simulink model "ACC4_FFNN_trainbfg_15_15_15_ep_100_Nor_20250527"  (R2021a)
settings: Solver=FixedStepAuto  StartTime=0.0  StopTime=T  RelTol=1e-3
undefined symbols (not defined in the file or in its folder): t_gap, Ts, v0_ego, v0_lead, v_set, x0_ego, x0_lead, x_gain, x_offset, y_gain, y_offset
libraries: neural x50
(part 2 of 2)

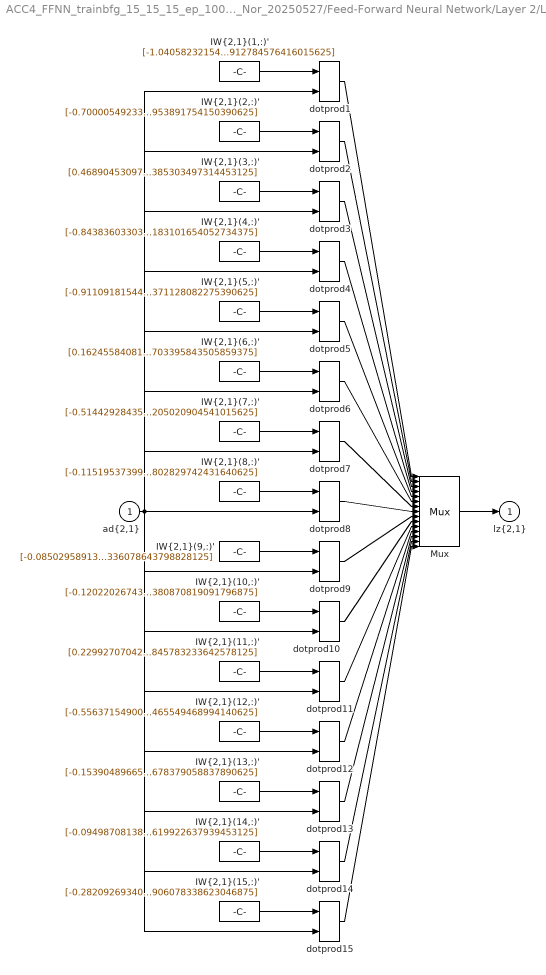
== system ACC4_FFNN_trainbfg_15_15_15_ep_100_Nor_20250527/Feed-Forward Neural Network/Layer 2/LW{2,1} ==
  "ad{2,1}" : Inport  PortDimensions=15
      mask Display: e = 0.06;c1 = [120 230 180]/255;c2 = ([120 230 180]+0)/(256+128);c3 = ([120 230 180]+128)/(256+128);patch([0 1 1 0],[0 0 1 1],c1);patch([0 1 1 1-e 1-e 0+e],[0 0 1 1-e 0+e 0+e],c2);patch([0 0 1 1-e 0+e 0+e],[0 1 1 1-e 1-e 0+e],c3);plot([0 1 1 0 0],[0 0 1 1 0]);
  "IW{2,1}(1,:)'" : Constant  Value=[-1.0405823215489833355462678809999488294124603271484375;-0.9608271683105680249781244128826074302196502685546875;0.5476392940007086540532554863602854311466217041015625;-0.1860903257221864226522711760480888187885284423828125;0.70133754923509872281073285193997435271739959716796875;-0.54431412858791627940036050858907401561737060546875;0.5380581706717924017624454791075550019741058349609375;-0.9009348419158775822523921306128613650798797607421875;-0.7521354448038597428904949993011541664600372314453125;0.241917287870616615208518851432017982006072998046875;-0.7321374980240575869316899115801788866519927978515625;-0.6457849324217816988635831876308657228946685791015625;-0.64376602939558436045075495712808333337306976318359375;-0.63161180496894697711240951321087777614593505859375;0.516510433268904112225072822184301912784576416015625]
      mask Display: e = 0.06;c1 = [120 150 230]/255;c2 = ([120 150 230]+0)/383;c3 = ([120 150 230]+128)/383;patch([0 1 1 0],[0 0 1 1],c1);patch([0 1 1 1-e 1-e 0+e],[0 0 1 1-e 0+e 0+e],c2);patch([0 0 1 1-e 0+e 0+e],[0 1 1 1-e 1-e 0+e],c3);plot([0 1 1 0 0],[0 0 1 1 0]);disp('weights');
  "IW{2,1}(10,:)'" : Constant  Value=[-0.120220267431918659273293314981856383383274078369140625;0.5302574432542292992565080567146651446819305419921875;1.0844112018206886194349181096185930073261260986328125;0.3573046096003764660054002888500690460205078125;0.73117639412220347683302179575548507273197174072265625;-0.75418929339658602462037606528610922396183013916015625;-0.581189831958130564970588238793425261974334716796875;-0.4362662882391401542037101535242982208728790283203125;-0.588048968935513283184945976245217025279998779296875;0.968796624481943258189176049199886620044708251953125;0.6844132248386689543195871010539121925830841064453125;-0.3617435753298094969210296767414547502994537353515625;-0.00872169059706992023939253755315803573466837406158447265625;-0.1165558858711521761364338090061210095882415771484375;0.36089370267177389717261348778265528380870819091796875]
      mask Display: e = 0.06;c1 = [120 150 230]/255;c2 = ([120 150 230]+0)/383;c3 = ([120 150 230]+128)/383;patch([0 1 1 0],[0 0 1 1],c1);patch([0 1 1 1-e 1-e 0+e],[0 0 1 1-e 0+e 0+e],c2);patch([0 0 1 1-e 0+e 0+e],[0 1 1 1-e 1-e 0+e],c3);plot([0 1 1 0 0],[0 0 1 1 0]);disp('weights');
  "IW{2,1}(11,:)'" : Constant  Value=[0.2299270704222209360523265786468982696533203125;-0.1990641851978147414126141256929258815944194793701171875;0.0157493935539519784583273320777152548544108867645263671875;-0.0096459618206787833827320355339907109737396240234375;0.225314821626530104037300361596862785518169403076171875;0.1739138266543526489815718605314032174646854400634765625;0.1045826830775500315695580866304226219654083251953125;0.07719335609068078696282100281678140163421630859375;0.8958662425863372913426019295002333819866180419921875;0.7178776333677323595594543803599663078784942626953125;0.118065089977390069719831444672308862209320068359375;-0.23311728925552344104943358615855686366558074951171875;0.7705319447275733590885238299961201846599578857421875;-0.97343359906549498106187456869520246982574462890625;0.043267329398776928350844883652825956232845783233642578125]
      mask Display: e = 0.06;c1 = [120 150 230]/255;c2 = ([120 150 230]+0)/383;c3 = ([120 150 230]+128)/383;patch([0 1 1 0],[0 0 1 1],c1);patch([0 1 1 1-e 1-e 0+e],[0 0 1 1-e 0+e 0+e],c2);patch([0 0 1 1-e 0+e 0+e],[0 1 1 1-e 1-e 0+e],c3);plot([0 1 1 0 0],[0 0 1 1 0]);disp('weights');
  "IW{2,1}(12,:)'" : Constant  Value=[-0.556371549001076548535138499573804438114166259765625;0.6163768674988137075132499376195482909679412841796875;0.454735929886855572146231452279607765376567840576171875;-0.6205791879648396847102276296936906874179840087890625;0.9799003554114114056261541918502189218997955322265625;0.10021329629212542833283094978469307534396648406982421875;0.25976677012884241690926501178182661533355712890625;0.390326078888663996480090645491145551204681396484375;-0.835857585804548275376646415679715573787689208984375;0.571117978530061076725132807041518390178680419921875;0.70819989854688625285916714346967637538909912109375;-0.246601959183730790048372227829531766474246978759765625;-0.94243259499025811010142206214368343353271484375;0.794382701947144109766441033571027219295501708984375;-0.89798245506530138815293184961774386465549468994140625]
      mask Display: e = 0.06;c1 = [120 150 230]/255;c2 = ([120 150 230]+0)/383;c3 = ([120 150 230]+128)/383;patch([0 1 1 0],[0 0 1 1],c1);patch([0 1 1 1-e 1-e 0+e],[0 0 1 1-e 0+e 0+e],c2);patch([0 0 1 1-e 0+e 0+e],[0 1 1 1-e 1-e 0+e],c3);plot([0 1 1 0 0],[0 0 1 1 0]);disp('weights');
  "IW{2,1}(13,:)'" : Constant  Value=[-0.153904896659829371063921144013875164091587066650390625;0.5090717228071948152745562765630893409252166748046875;-0.29697183815985350729960146054509095847606658935546875;-0.0099883500195583341252358877682127058506011962890625;0.05536005484219876093821000040406943298876285552978515625;0.1251542077321984580695612976342090405523777008056640625;-0.9360179684748661799176261411048471927642822265625;-0.0017679730348210132007125139352865517139434814453125;-0.7885811468365571119676360467565245926380157470703125;0.0267548371751498148540804322692565619945526123046875;-0.3042416113454777804037121313740499317646026611328125;0.261979220371351961826889009898877702653408050537109375;0.2643737023407515263073719324893318116664886474609375;-0.606683617264736074758957329322583973407745361328125;-0.95567583042114601088456993238651193678379058837890625]
      mask Display: e = 0.06;c1 = [120 150 230]/255;c2 = ([120 150 230]+0)/383;c3 = ([120 150 230]+128)/383;patch([0 1 1 0],[0 0 1 1],c1);patch([0 1 1 1-e 1-e 0+e],[0 0 1 1-e 0+e 0+e],c2);patch([0 0 1 1-e 0+e 0+e],[0 1 1 1-e 1-e 0+e],c3);plot([0 1 1 0 0],[0 0 1 1 0]);disp('weights');
  "IW{2,1}(14,:)'" : Constant  Value=[-0.0949870813828463667061186015416751615703105926513671875;-0.230612941886796762869238364146440289914608001708984375;-1.0507342618771271514077625397476367652416229248046875;-0.7047835560466226834108738330542109906673431396484375;-0.04152563470139190859864442018078989349305629730224609375;0.58730051068405131342586855680565349757671356201171875;0.2294268382342810053131643144297413527965545654296875;0.071602111502226506445367704145610332489013671875;-0.7159177561920035959275310233351774513721466064453125;-0.644795078988269931841159632313065230846405029296875;-0.1079467038897943265141066149226389825344085693359375;0.48203925309316908442980320614879019558429718017578125;0.33818146513637958872067201809841208159923553466796875;-0.8132589664898139947268873584107495844364166259765625;0.478036667924507885363283321566996164619922637939453125]
      mask Display: e = 0.06;c1 = [120 150 230]/255;c2 = ([120 150 230]+0)/383;c3 = ([120 150 230]+128)/383;patch([0 1 1 0],[0 0 1 1],c1);patch([0 1 1 1-e 1-e 0+e],[0 0 1 1-e 0+e 0+e],c2);patch([0 0 1 1-e 0+e 0+e],[0 1 1 1-e 1-e 0+e],c3);plot([0 1 1 0 0],[0 0 1 1 0]);disp('weights');
  "IW{2,1}(15,:)'" : Constant  Value=[-0.2820926934058338719779612802085466682910919189453125;-0.55856947057804762213351068567135371267795562744140625;-0.551556482284416116357306236750446259975433349609375;-0.890051706187623636878925026394426822662353515625;0.60240233369460483014989904404501430690288543701171875;0.96460639263537995002906200170400552451610565185546875;-0.2751770754538946928136056158109568059444427490234375;-0.10963366940791541281896570581011474132537841796875;-0.667079118247158486809667010675184428691864013671875;-0.2028210065283138074931912342435680329799652099609375;-0.891521031117740836435814344440586864948272705078125;-0.799556919609016869543438588152639567852020263671875;0.12267233388357355605702281309277168475091457366943359375;-0.3852662008241598545765782546368427574634552001953125;0.6905806241987288984773840638808906078338623046875]
      mask Display: e = 0.06;c1 = [120 150 230]/255;c2 = ([120 150 230]+0)/383;c3 = ([120 150 230]+128)/383;patch([0 1 1 0],[0 0 1 1],c1);patch([0 1 1 1-e 1-e 0+e],[0 0 1 1-e 0+e 0+e],c2);patch([0 0 1 1-e 0+e 0+e],[0 1 1 1-e 1-e 0+e],c3);plot([0 1 1 0 0],[0 0 1 1 0]);disp('weights');
  "IW{2,1}(2,:)'" : Constant  Value=[-0.7000054923366338943679920703289099037647247314453125;-0.3382842395718579364682909726980142295360565185546875;0.8986078236995937995601479997276328504085540771484375;0.4974114364313828584585053249611519277095794677734375;0.1211190547097695802136740894638933241367340087890625;-0.003811417607220590753058786503970623016357421875;0.162892975750795532263737186440266668796539306640625;-0.0208600216453564968333012075163424015045166015625;-0.0192854130639636967003980316803790628910064697265625;0.147419529682396355241280616610310971736907958984375;-0.9382209025100969324029165363754145801067352294921875;0.325616123921948830144401654251851141452789306640625;-0.2807301730358393587749787911889143288135528564453125;0.19442270067570976976867314078845083713531494140625;-0.7966612127504897333807321047061122953891754150390625]
      mask Display: e = 0.06;c1 = [120 150 230]/255;c2 = ([120 150 230]+0)/383;c3 = ([120 150 230]+128)/383;patch([0 1 1 0],[0 0 1 1],c1);patch([0 1 1 1-e 1-e 0+e],[0 0 1 1-e 0+e 0+e],c2);patch([0 0 1 1-e 0+e 0+e],[0 1 1 1-e 1-e 0+e],c3);plot([0 1 1 0 0],[0 0 1 1 0]);disp('weights');
  "IW{2,1}(3,:)'" : Constant  Value=[0.46890453097095063927923774826922453939914703369140625;-0.1600608568250439234237347818634589202702045440673828125;-0.12399845995805358622732228468521498143672943115234375;0.6511676315723111674316214703139849007129669189453125;0.85938165041460357063130004462436772882938385009765625;0.967936511731725790497193884220905601978302001953125;0.856626124628375951175485170097090303897857666015625;-0.6149792078758504754176783535513095557689666748046875;0.7059963106816324884817959173233248293399810791015625;-0.8958442194282607573541099554859101772308349609375;0.8782834121390958870279064285568892955780029296875;-0.206000980504430941664395504631102085113525390625;-0.77406206789949927316030198198859579861164093017578125;-0.4001260198204221740780894833733327686786651611328125;0.82207842077581905204652912289020605385303497314453125]
      mask Display: e = 0.06;c1 = [120 150 230]/255;c2 = ([120 150 230]+0)/383;c3 = ([120 150 230]+128)/383;patch([0 1 1 0],[0 0 1 1],c1);patch([0 1 1 1-e 1-e 0+e],[0 0 1 1-e 0+e 0+e],c2);patch([0 0 1 1-e 0+e 0+e],[0 1 1 1-e 1-e 0+e],c3);plot([0 1 1 0 0],[0 0 1 1 0]);disp('weights');
  "IW{2,1}(4,:)'" : Constant  Value=[-0.84383603303488075031424386907019652426242828369140625;-0.45965468593376723749344137104344554245471954345703125;0.0104593103155407908533280902929618605412542819976806640625;0.579926059889061651375641304184682667255401611328125;0.3933344011104551452007171974400989711284637451171875;-0.08418835848849438863172878200202831067144870758056640625;0.1601807315168832790419628508971072733402252197265625;-0.753832504908109601871046834276057779788970947265625;0.7478548117234666836594669803162105381488800048828125;0.862402769216499276438980814418755471706390380859375;-0.3973878708272156057290658281999640166759490966796875;0.6115292870810014047577851670212112367153167724609375;-0.11578681594154351108816314308569417335093021392822265625;-0.7317541343426352540291190962307155132293701171875;-0.417232981103956512836106185204698704183101654052734375]
      mask Display: e = 0.06;c1 = [120 150 230]/255;c2 = ([120 150 230]+0)/383;c3 = ([120 150 230]+128)/383;patch([0 1 1 0],[0 0 1 1],c1);patch([0 1 1 1-e 1-e 0+e],[0 0 1 1-e 0+e 0+e],c2);patch([0 0 1 1-e 0+e 0+e],[0 1 1 1-e 1-e 0+e],c3);plot([0 1 1 0 0],[0 0 1 1 0]);disp('weights');
  "IW{2,1}(5,:)'" : Constant  Value=[-0.9110918154435230231769082820392213761806488037109375;-0.6058924038090884867102658972726203501224517822265625;-0.122710034826088776327424056944437325000762939453125;-0.3629515092020156874497160970349796116352081298828125;0.165581930351680117752266596653498709201812744140625;0.6903563701080732695203323601162992417812347412109375;-0.96603412332547744512112330994568765163421630859375;-0.5890116581846402965538800344802439212799072265625;-0.45941133541460477118789640371687710285186767578125;0.457323363356542333946208600536920130252838134765625;-0.408932331049287167701322687207721173763275146484375;-0.763689603106578740465693044825457036495208740234375;-0.3283020506461509224749306667945347726345062255859375;-0.574796933282314181923311480204574763774871826171875;-0.4053063682241566656472286922507919371128082275390625]
      mask Display: e = 0.06;c1 = [120 150 230]/255;c2 = ([120 150 230]+0)/383;c3 = ([120 150 230]+128)/383;patch([0 1 1 0],[0 0 1 1],c1);patch([0 1 1 1-e 1-e 0+e],[0 0 1 1-e 0+e 0+e],c2);patch([0 0 1 1-e 0+e 0+e],[0 1 1 1-e 1-e 0+e],c3);plot([0 1 1 0 0],[0 0 1 1 0]);disp('weights');
  "IW{2,1}(6,:)'" : Constant  Value=[0.162455840818920560497673477584612555801868438720703125;0.642616637081111274909517305786721408367156982421875;0.350996130621946067495997567675658501684665679931640625;0.0681282547414527872575717992731370031833648681640625;0.63079436754187601099630455792066641151905059814453125;0.253691470335771274147163012457895092666149139404296875;-0.7582808578028836787865429869270883500576019287109375;-0.7069701787702202810947937905439175665378570556640625;-0.5830772824973724510755346273072063922882080078125;0.4756833075951802936032208890537731349468231201171875;-0.3341274363276494074881384221953339874744415283203125;0.7989442886824651424149124068208038806915283203125;-0.800060224384415707987727728323079645633697509765625;0.789883350881628754081020815647207200527191162109375;-0.95452869287727748481842127148411236703395843505859375]
      mask Display: e = 0.06;c1 = [120 150 230]/255;c2 = ([120 150 230]+0)/383;c3 = ([120 150 230]+128)/383;patch([0 1 1 0],[0 0 1 1],c1);patch([0 1 1 1-e 1-e 0+e],[0 0 1 1-e 0+e 0+e],c2);patch([0 0 1 1-e 0+e 0+e],[0 1 1 1-e 1-e 0+e],c3);plot([0 1 1 0 0],[0 0 1 1 0]);disp('weights');
  "IW{2,1}(7,:)'" : Constant  Value=[-0.5144292843580762220057067679590545594692230224609375;-0.140157181233467209580112466937862336635589599609375;0.537708504859229829975220127380453050136566162109375;-0.82009864245883790090374532155692577362060546875;0.7580278091943555285325828663189895451068878173828125;0.17197407165295164332974309218116104602813720703125;0.725421437399339286145050209597684442996978759765625;-0.621855651054772362584799338947050273418426513671875;0.1299591414764023067363041263888590037822723388671875;-0.8731909986143635560296161202131770551204681396484375;-0.065863625942295112025703929248265922069549560546875;0.0799641980758583059696320560760796070098876953125;-0.582106652013729242156614418490789830684661865234375;-0.8570943744259109653427231023670174181461334228515625;-0.40351205622447228194005219847895205020904541015625]
      mask Display: e = 0.06;c1 = [120 150 230]/255;c2 = ([120 150 230]+0)/383;c3 = ([120 150 230]+128)/383;patch([0 1 1 0],[0 0 1 1],c1);patch([0 1 1 1-e 1-e 0+e],[0 0 1 1-e 0+e 0+e],c2);patch([0 0 1 1-e 0+e 0+e],[0 1 1 1-e 1-e 0+e],c3);plot([0 1 1 0 0],[0 0 1 1 0]);disp('weights');
  "IW{2,1}(8,:)'" : Constant  Value=[-0.1151953739961133482694322083261795341968536376953125;0.7755419085127075451424616403528489172458648681640625;-0.665492909010556576987482912954874336719512939453125;-0.776588511613593102111963162315078079700469970703125;0.9778232321591782127967462656670249998569488525390625;-0.5065309480280502096860573146841488778591156005859375;-0.031406977575795025359184364788234233856201171875;-0.9146951781777132861606105507235042750835418701171875;0.2806236503255161718328736242256127297878265380859375;0.720881126076463818463935240288265049457550048828125;0.2963968129323142353115372316096909344196319580078125;0.413834838645525504574607111862860620021820068359375;0.8103071180089280733938039702479727566242218017578125;-0.5150268821265611141058116118074394762516021728515625;-0.90729747020363848974966458627022802829742431640625]
      mask Display: e = 0.06;c1 = [120 150 230]/255;c2 = ([120 150 230]+0)/383;c3 = ([120 150 230]+128)/383;patch([0 1 1 0],[0 0 1 1],c1);patch([0 1 1 1-e 1-e 0+e],[0 0 1 1-e 0+e 0+e],c2);patch([0 0 1 1-e 0+e 0+e],[0 1 1 1-e 1-e 0+e],c3);plot([0 1 1 0 0],[0 0 1 1 0]);disp('weights');
  "IW{2,1}(9,:)'" : Constant  Value=[-0.08502958913522730421963302660515182651579380035400390625;-0.2182372384019506117436293379796552471816539764404296875;0.309604443959900610394697650917805731296539306640625;-0.727414902123402651312744637834839522838592529296875;-0.99895538327737021244701054456527344882488250732421875;0.045954384797662332917678185140175628475844860076904296875;0.6897113491525264095116654061712324619293212890625;0.270395833719764056013445951975882053375244140625;-0.16594209671422799345918974722735583782196044921875;0.8688102379224267313162499704048968851566314697265625;-0.9495436370139274107060600726981647312641143798828125;0.77107377246475639065437235331046395003795623779296875;0.15514524096584392243158845303696580231189727783203125;-0.892491215582572383624437861726619303226470947265625;-0.1202330084681953181746649761407752521336078643798828125]
      mask Display: e = 0.06;c1 = [120 150 230]/255;c2 = ([120 150 230]+0)/383;c3 = ([120 150 230]+128)/383;patch([0 1 1 0],[0 0 1 1],c1);patch([0 1 1 1-e 1-e 0+e],[0 0 1 1-e 0+e 0+e],c2);patch([0 0 1 1-e 0+e 0+e],[0 1 1 1-e 1-e 0+e],c3);plot([0 1 1 0 0],[0 0 1 1 0]);disp('weights');
  Mux : Mux  Inputs=15
      mask Display: e = 0.06;c1 = [120 150 230]/255;c2 = ([120 150 230]+0)/383;c3 = ([120 150 230]+128)/383;patch([0 1 1 0],[0 0 1 1],c1);patch([0 1 1 1-e 1-e 0+e],[0 0 1 1-e 0+e 0+e],c2);patch([0 0 1 1-e 0+e 0+e],[0 1 1 1-e 1-e 0+e],c3);plot([0 1 1 0 0],[0 0 1 1 0]);disp('Mux');
  dotprod{1..15} (15 alike) : neural/Weight Functions/dotprod
  "lz{2,1}" : Outport
      mask Display: e = 0.06;c1 = [120 230 180]/255;c2 = ([120 230 180]+0)/(256+128);c3 = ([120 230 180]+128)/(256+128);patch([0 1 1 0],[0 0 1 1],c1);patch([0 1 1 1-e 1-e 0+e],[0 0 1 1-e 0+e 0+e],c2);patch([0 0 1 1-e 0+e 0+e],[0 1 1 1-e 1-e 0+e],c3);plot([0 1 1 0 0],[0 0 1 1 0]);
  wires:
  Mux/1 -> "lz{2,1}"/1
  dotprod15/1 -> Mux/15
  "IW{2,1}(15,:)'"/1 -> dotprod15/1
  dotprod14/1 -> Mux/14
  "IW{2,1}(14,:)'"/1 -> dotprod14/1
  dotprod13/1 -> Mux/13
  "IW{2,1}(13,:)'"/1 -> dotprod13/1
  dotprod12/1 -> Mux/12
  "IW{2,1}(12,:)'"/1 -> dotprod12/1
  dotprod11/1 -> Mux/11
  "IW{2,1}(11,:)'"/1 -> dotprod11/1
  dotprod10/1 -> Mux/10
  "IW{2,1}(10,:)'"/1 -> dotprod10/1
  dotprod9/1 -> Mux/9
  "IW{2,1}(9,:)'"/1 -> dotprod9/1
  dotprod8/1 -> Mux/8
  "IW{2,1}(8,:)'"/1 -> dotprod8/1
  dotprod7/1 -> Mux/7
  "IW{2,1}(7,:)'"/1 -> dotprod7/1
  dotprod6/1 -> Mux/6
  "IW{2,1}(6,:)'"/1 -> dotprod6/1
  dotprod5/1 -> Mux/5
  "IW{2,1}(5,:)'"/1 -> dotprod5/1
  dotprod4/1 -> Mux/4
  "IW{2,1}(4,:)'"/1 -> dotprod4/1
  dotprod3/1 -> Mux/3
  "IW{2,1}(3,:)'"/1 -> dotprod3/1
  dotprod2/1 -> Mux/2
  "IW{2,1}(2,:)'"/1 -> dotprod2/1
  dotprod1/1 -> Mux/1
  "ad{2,1}"/1 -> dotprod15/2, dotprod14/2, dotprod13/2, dotprod12/2, dotprod11/2, dotprod10/2, dotprod9/2, dotprod8/2, dotprod7/2, dotprod6/2, dotprod5/2, dotprod4/2, dotprod3/2, dotprod2/2, dotprod1/2
  "IW{2,1}(1,:)'"/1 -> dotprod1/1

== system ACC4_FFNN_trainbfg_15_15_15_ep_100_Nor_20250527/Feed-Forward Neural Network/Layer 3/Delays 1 ==
  "p{3}" : Inport  PortDimensions=15
      mask Display: e = 0.06;c1 = [120 230 180]/255;c2 = ([120 230 180]+0)/(256+128);c3 = ([120 230 180]+128)/(256+128);patch([0 1 1 0],[0 0 1 1],c1);patch([0 1 1 1-e 1-e 0+e],[0 0 1 1-e 0+e 0+e],c2);patch([0 0 1 1-e 0+e 0+e],[0 1 1 1-e 1-e 0+e],c3);plot([0 1 1 0 0],[0 0 1 1 0]);
  mux : Mux  Inputs=1
      mask Display: e = 0.06;c1 = [120 150 230]/255;c2 = ([120 150 230]+0)/383;c3 = ([120 150 230]+128)/383;patch([0 1 1 0],[0 0 1 1],c1);patch([0 1 1 1-e 1-e 0+e],[0 0 1 1-e 0+e 0+e],c2);patch([0 0 1 1-e 0+e 0+e],[0 1 1 1-e 1-e 0+e],c3);plot([0 1 1 0 0],[0 0 1 1 0]);disp('Mux')
  "pd{3,2}" : Outport
      mask Display: e = 0.06;c1 = [120 230 180]/255;c2 = ([120 230 180]+0)/(256+128);c3 = ([120 230 180]+128)/(256+128);patch([0 1 1 0],[0 0 1 1],c1);patch([0 1 1 1-e 1-e 0+e],[0 0 1 1-e 0+e 0+e],c2);patch([0 0 1 1-e 0+e 0+e],[0 1 1 1-e 1-e 0+e],c3);plot([0 1 1 0 0],[0 0 1 1 0]);
  wires:
  mux/1 -> "pd{3,2}"/1
  "p{3}"/1 -> mux/1

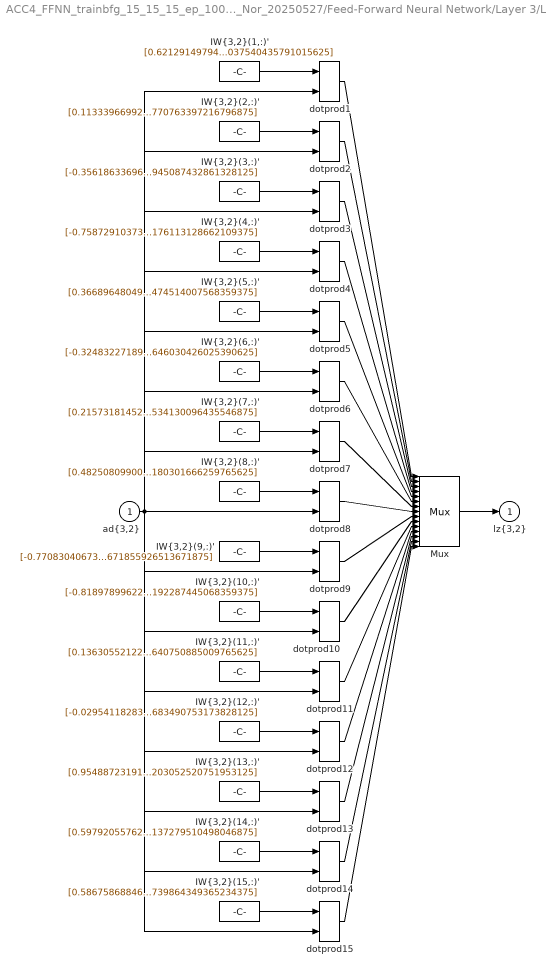
== system ACC4_FFNN_trainbfg_15_15_15_ep_100_Nor_20250527/Feed-Forward Neural Network/Layer 3/LW{3,2} ==
  "ad{3,2}" : Inport  PortDimensions=15
      mask Display: e = 0.06;c1 = [120 230 180]/255;c2 = ([120 230 180]+0)/(256+128);c3 = ([120 230 180]+128)/(256+128);patch([0 1 1 0],[0 0 1 1],c1);patch([0 1 1 1-e 1-e 0+e],[0 0 1 1-e 0+e 0+e],c2);patch([0 0 1 1-e 0+e 0+e],[0 1 1 1-e 1-e 0+e],c3);plot([0 1 1 0 0],[0 0 1 1 0]);
  "IW{3,2}(1,:)'" : Constant  Value=[0.6212914979485184563401389823411591351032257080078125;-0.897336227775257899708094555535353720188140869140625;0.2520710676594088983648589419317431747913360595703125;-0.61253412590856959329954634085879661142826080322265625;-0.7754320756879466980393544872640632092952728271484375;-0.408881094741323003471933361652190797030925750732421875;-0.81529532256159686909313677460886538028717041015625;-0.367142001707418064171406513196416199207305908203125;0.5050408928388991913749350715079344809055328369140625;-0.473339240559633001037553867718088440597057342529296875;-0.94785817441970243724114197902963496744632720947265625;-0.1580605200614016159210706291560200043022632598876953125;0.316865218257510627974937733597471378743648529052734375;0.63161547925595817876143200919614173471927642822265625;-0.1548218243703395613497519889278919436037540435791015625]
      mask Display: e = 0.06;c1 = [120 150 230]/255;c2 = ([120 150 230]+0)/383;c3 = ([120 150 230]+128)/383;patch([0 1 1 0],[0 0 1 1],c1);patch([0 1 1 1-e 1-e 0+e],[0 0 1 1-e 0+e 0+e],c2);patch([0 0 1 1-e 0+e 0+e],[0 1 1 1-e 1-e 0+e],c3);plot([0 1 1 0 0],[0 0 1 1 0]);disp('weights');
  "IW{3,2}(10,:)'" : Constant  Value=[-0.81897899622015579712552835189853794872760772705078125;-0.7650142956963341678289225455955602228641510009765625;0.210079761258290809156079603781108744442462921142578125;-0.411867332482743098154287508805282413959503173828125;0.3109960796070747601760331235709600150585174560546875;-0.8811934062834456682367090252228081226348876953125;-0.731393391372850754095225056516937911510467529296875;0.8276008215591357242146841599605977535247802734375;0.241374790756772539257468679352314211428165435791015625;-0.1116963821918613153361121703710523433983325958251953125;0.55277095995546721152180680292076431214809417724609375;0.4054046139009506166672736071632243692874908447265625;-0.489226519023898465121646950137801468372344970703125;0.33623442737450670581011991089326329529285430908203125;0.6523830987678420623154806889942847192287445068359375]
      mask Display: e = 0.06;c1 = [120 150 230]/255;c2 = ([120 150 230]+0)/383;c3 = ([120 150 230]+128)/383;patch([0 1 1 0],[0 0 1 1],c1);patch([0 1 1 1-e 1-e 0+e],[0 0 1 1-e 0+e 0+e],c2);patch([0 0 1 1-e 0+e 0+e],[0 1 1 1-e 1-e 0+e],c3);plot([0 1 1 0 0],[0 0 1 1 0]);disp('weights');
  "IW{3,2}(11,:)'" : Constant  Value=[0.1363055212215608380521558729014941491186618804931640625;0.2814358459318511140878626974881626665592193603515625;0.51267928560415920724580018941196613013744354248046875;-0.5252539605888415508161415345966815948486328125;-0.780489898553896832567033925442956387996673583984375;-0.3683771233222679075680616733734495937824249267578125;-0.8028118145780045455950357791152782738208770751953125;0.4134304353938611509278189259930513799190521240234375;-0.6912726051021162998466706994804553687572479248046875;-0.306343189844245966657609869798761792480945587158203125;0.494689388045416345018878701011999510228633880615234375;-0.692819246761199547535170495393685996532440185546875;-0.9589284506836308619170949896215461194515228271484375;0.402843052338233587050808637286536395549774169921875;0.2798823085962445222918404397205449640750885009765625]
      mask Display: e = 0.06;c1 = [120 150 230]/255;c2 = ([120 150 230]+0)/383;c3 = ([120 150 230]+128)/383;patch([0 1 1 0],[0 0 1 1],c1);patch([0 1 1 1-e 1-e 0+e],[0 0 1 1-e 0+e 0+e],c2);patch([0 0 1 1-e 0+e 0+e],[0 1 1 1-e 1-e 0+e],c3);plot([0 1 1 0 0],[0 0 1 1 0]);disp('weights');
  "IW{3,2}(12,:)'" : Constant  Value=[-0.029541182830081336163630112423561513423919677734375;-0.342371570486394549703845768817700445652008056640625;-0.415317728776301964277450906593003310263156890869140625;0.02038573702696593048511175538806128315627574920654296875;0.86751969677066487207639511325396597385406494140625;-0.11968676677248414608190074659432866610586643218994140625;-0.7159455031361432464365179839660413563251495361328125;0.1155779335097524285203007821110077202320098876953125;-1.0525364076032477367306228188681416213512420654296875;0.0935068596179075284258175315699190832674503326416015625;0.08389729679892454772272003538091666996479034423828125;0.760443009673319902930188618483953177928924560546875;0.32516639881796371991384830835158936679363250732421875;-0.1987915137881836880051622529208543710410594940185546875;-0.2898526962423020325587685874779708683490753173828125]
      mask Display: e = 0.06;c1 = [120 150 230]/255;c2 = ([120 150 230]+0)/383;c3 = ([120 150 230]+128)/383;patch([0 1 1 0],[0 0 1 1],c1);patch([0 1 1 1-e 1-e 0+e],[0 0 1 1-e 0+e 0+e],c2);patch([0 0 1 1-e 0+e 0+e],[0 1 1 1-e 1-e 0+e],c3);plot([0 1 1 0 0],[0 0 1 1 0]);disp('weights');
  "IW{3,2}(13,:)'" : Constant  Value=[0.95488723191072544249635711821611039340496063232421875;0.3076240451915472906563309152261354029178619384765625;-0.593435468543333843882692235638387501239776611328125;-0.78574984872688158343834174957009963691234588623046875;-0.62507838715662700224129366688430309295654296875;0.9310703838417444533348543700412847101688385009765625;-0.6634974030169444869642347839544527232646942138671875;-0.3731420201268174086095541497343219816684722900390625;-0.0187368953208103504459725030528716160915791988372802734375;0.377012564358657709107092159683816134929656982421875;0.73299533791845383756680121223325841128826141357421875;0.20020005042144728424347022155416198074817657470703125;0.7305624294098811422060180120752193033695220947265625;0.1976499640218950804015918265577056445181369781494140625;1.1481278185603660535463177438941784203052520751953125]
      mask Display: e = 0.06;c1 = [120 150 230]/255;c2 = ([120 150 230]+0)/383;c3 = ([120 150 230]+128)/383;patch([0 1 1 0],[0 0 1 1],c1);patch([0 1 1 1-e 1-e 0+e],[0 0 1 1-e 0+e 0+e],c2);patch([0 0 1 1-e 0+e 0+e],[0 1 1 1-e 1-e 0+e],c3);plot([0 1 1 0 0],[0 0 1 1 0]);disp('weights');
  "IW{3,2}(14,:)'" : Constant  Value=[0.597920557625758686270955877262167632579803466796875;0.498262926207038159276407895958982408046722412109375;-0.8266669052089354874368609671364538371562957763671875;-0.189369160238817446639814079389907419681549072265625;-0.4676423221847223476999033664469607174396514892578125;-0.7493356377816400293312426583725027740001678466796875;-0.6075021554860893235883168017608113586902618408203125;-0.6675928741956986822714270601863972842693328857421875;0.516224862654837135522711832891218364238739013671875;-0.1513304327486186817708357921219430863857269287109375;-0.7881591665344693797834452198003418743610382080078125;0.3594677964209338494327994339982978999614715576171875;0.8652271440971281979415152818546630442142486572265625;-0.2184758355916509575678219334804452955722808837890625;-0.551657002033745680336096484097652137279510498046875]
      mask Display: e = 0.06;c1 = [120 150 230]/255;c2 = ([120 150 230]+0)/383;c3 = ([120 150 230]+128)/383;patch([0 1 1 0],[0 0 1 1],c1);patch([0 1 1 1-e 1-e 0+e],[0 0 1 1-e 0+e 0+e],c2);patch([0 0 1 1-e 0+e 0+e],[0 1 1 1-e 1-e 0+e],c3);plot([0 1 1 0 0],[0 0 1 1 0]);disp('weights');
  "IW{3,2}(15,:)'" : Constant  Value=[0.5867586884646709410873199885827489197254180908203125;0.1663714629097523545198100691777653992176055908203125;0.46617235130520950914245759122422896325588226318359375;-0.76905121362304551535515884097549133002758026123046875;0.5956605204231941730341759466682560741901397705078125;-0.397853832267614004880584843704127706587314605712890625;-0.36504044970112925483363142120651900768280029296875;0.244994518559790375178408794454298913478851318359375;1.1611614719548717378216906581656076014041900634765625;-0.2411508577944020681460557398168020881712436676025390625;0.49773332967986672059623742825351655483245849609375;-0.8515953082966631892958275784621946513652801513671875;-0.40459901921300278626603130760486237704753875732421875;0.8286805263588739034474883737857453525066375732421875;0.399824525098690486402119859121739864349365234375]
      mask Display: e = 0.06;c1 = [120 150 230]/255;c2 = ([120 150 230]+0)/383;c3 = ([120 150 230]+128)/383;patch([0 1 1 0],[0 0 1 1],c1);patch([0 1 1 1-e 1-e 0+e],[0 0 1 1-e 0+e 0+e],c2);patch([0 0 1 1-e 0+e 0+e],[0 1 1 1-e 1-e 0+e],c3);plot([0 1 1 0 0],[0 0 1 1 0]);disp('weights');
  "IW{3,2}(2,:)'" : Constant  Value=[0.1133396699280251329611246546846814453601837158203125;-0.854229401802047760838831891305744647979736328125;-0.530346170504191416483763532596640288829803466796875;-0.2234567379043965740237354111741296947002410888671875;0.5688557814878254514923128226655535399913787841796875;0.5379165281177382684774102017399854958057403564453125;-0.9843594128613302185470956828794442117214202880859375;-0.564873381154358700229067835607565939426422119140625;-0.6591359538862333611319854753674007952213287353515625;0.3710714174950744403957969552720896899700164794921875;-0.951131967899252028786349910660646855831146240234375;-0.5756735894901312544646998503594659268856048583984375;0.4972377435523942512674011595663614571094512939453125;0.589315770777506298117032201844267547130584716796875;0.6290795458013025420740405024844221770763397216796875]
      mask Display: e = 0.06;c1 = [120 150 230]/255;c2 = ([120 150 230]+0)/383;c3 = ([120 150 230]+128)/383;patch([0 1 1 0],[0 0 1 1],c1);patch([0 1 1 1-e 1-e 0+e],[0 0 1 1-e 0+e 0+e],c2);patch([0 0 1 1-e 0+e 0+e],[0 1 1 1-e 1-e 0+e],c3);plot([0 1 1 0 0],[0 0 1 1 0]);disp('weights');
  "IW{3,2}(3,:)'" : Constant  Value=[-0.356186336967777794626499598962254822254180908203125;-0.8229450806505591575756852762424387037754058837890625;0.54375825229309426855905940101365558803081512451171875;0.103557063914454960951161410775966942310333251953125;-0.416859364186138225960576164652593433856964111328125;-0.2079865095642496886085837104474194347858428955078125;-0.1537812296716669635543439653702080249786376953125;-0.4979163079685278159303152278880588710308074951171875;-0.484352604165497524491001968272030353546142578125;-0.27690400683290261607538695898256264626979827880859375;-0.35737529255803412997494206138071604073047637939453125;-0.8029625246237832580931126358336769044399261474609375;-0.7596259640258387069167156369076110422611236572265625;0.1587028832735242200868697182158939540386199951171875;0.407888275153397206196359547902829945087432861328125]
      mask Display: e = 0.06;c1 = [120 150 230]/255;c2 = ([120 150 230]+0)/383;c3 = ([120 150 230]+128)/383;patch([0 1 1 0],[0 0 1 1],c1);patch([0 1 1 1-e 1-e 0+e],[0 0 1 1-e 0+e 0+e],c2);patch([0 0 1 1-e 0+e 0+e],[0 1 1 1-e 1-e 0+e],c3);plot([0 1 1 0 0],[0 0 1 1 0]);disp('weights');
  "IW{3,2}(4,:)'" : Constant  Value=[-0.75872910373055357791116648513707332313060760498046875;0.5967017282279047929449689036118797957897186279296875;0.81184939659011201573690641453140415251255035400390625;-0.5420934959537999642265049260458908975124359130859375;0.207066877501773660696926526725292205810546875;-0.4541224117526188042148760359850712120532989501953125;0.3111463498758286760903501999564468860626220703125;0.785844810571953988898030729615129530429840087890625;-0.2064375506801996162931089884295943193137645721435546875;-0.0166521805415130695615655298524870886467397212982177734375;-0.4026578267676457212331797563820146024227142333984375;0.64714894785567711466001128428615629673004150390625;0.0500903295252175251306425707298330962657928466796875;-0.1413701702322114339693825968424789607524871826171875;0.75811962815322109232596403671777807176113128662109375]
      mask Display: e = 0.06;c1 = [120 150 230]/255;c2 = ([120 150 230]+0)/383;c3 = ([120 150 230]+128)/383;patch([0 1 1 0],[0 0 1 1],c1);patch([0 1 1 1-e 1-e 0+e],[0 0 1 1-e 0+e 0+e],c2);patch([0 0 1 1-e 0+e 0+e],[0 1 1 1-e 1-e 0+e],c3);plot([0 1 1 0 0],[0 0 1 1 0]);disp('weights');
  "IW{3,2}(5,:)'" : Constant  Value=[0.36689648049260636941681923417490907013416290283203125;0.8860162791414054606065064945141784846782684326171875;0.74274429969335298284960344972205348312854766845703125;0.283881240798374623324207277619279921054840087890625;0.928845334431802616137474615243263542652130126953125;-0.92553073185934398026120106806047260761260986328125;0.445845049384048675022995666950009763240814208984375;0.406446449112582097740187236922793090343475341796875;-0.851942647590646640054501403938047587871551513671875;0.7088576553696366300272302396479062736034393310546875;0.35616472828092204938599252272979356348514556884765625;-0.64998052523584082251772997551597654819488525390625;-0.3483327424735016553114519410883076488971710205078125;-0.48854493826714773252462009622831828892230987548828125;-0.19555835650756703270047864862135611474514007568359375]
      mask Display: e = 0.06;c1 = [120 150 230]/255;c2 = ([120 150 230]+0)/383;c3 = ([120 150 230]+128)/383;patch([0 1 1 0],[0 0 1 1],c1);patch([0 1 1 1-e 1-e 0+e],[0 0 1 1-e 0+e 0+e],c2);patch([0 0 1 1-e 0+e 0+e],[0 1 1 1-e 1-e 0+e],c3);plot([0 1 1 0 0],[0 0 1 1 0]);disp('weights');
  "IW{3,2}(6,:)'" : Constant  Value=[-0.3248322718959097965552018649759702384471893310546875;0.367431144816716237500031638774089515209197998046875;-0.9707858745819049062220074119977653026580810546875;-0.070374726122290842678097533280379138886928558349609375;-0.135030012059278003988538330304436385631561279296875;-0.2860024317113118996758203138597309589385986328125;0.0624185871648774703857043277821503579616546630859375;0.1114758854387731812352058113901875913143157958984375;-0.4071531019816105878561529607395641505718231201171875;0.17298045799577532743995789132895879447460174560546875;0.535914099683644895577572242473252117633819580078125;-0.81216581982098290382054983638226985931396484375;-0.4037402263156171233760005634394474327564239501953125;0.044604134995013970665933555892479489557445049285888671875;0.271322777722753816220802036696113646030426025390625]
      mask Display: e = 0.06;c1 = [120 150 230]/255;c2 = ([120 150 230]+0)/383;c3 = ([120 150 230]+128)/383;patch([0 1 1 0],[0 0 1 1],c1);patch([0 1 1 1-e 1-e 0+e],[0 0 1 1-e 0+e 0+e],c2);patch([0 0 1 1-e 0+e 0+e],[0 1 1 1-e 1-e 0+e],c3);plot([0 1 1 0 0],[0 0 1 1 0]);disp('weights');
  "IW{3,2}(7,:)'" : Constant  Value=[0.215731814525891518741218533250503242015838623046875;-0.735834088572874467359952177503146231174468994140625;-0.333401583857998728976923530353815294802188873291015625;-0.6963089497674668226778749158256687223911285400390625;0.3895043892358802661846084447461180388927459716796875;-0.14087108149629390396739836432971060276031494140625;-0.782364123453909154903840317274443805217742919921875;-0.631132664484693517437108312151394784450531005859375;-0.1952237065882627409241223404023912735283374786376953125;-0.35919164495900124389748953035450540482997894287109375;0.8543277768740187294582710819668136537075042724609375;0.3319744328222211660062157534412108361721038818359375;-0.20223849523360204472055556834675371646881103515625;-0.57199581590514991802365329931490123271942138671875;0.87488889348161347214727356913499534130096435546875]
      mask Display: e = 0.06;c1 = [120 150 230]/255;c2 = ([120 150 230]+0)/383;c3 = ([120 150 230]+128)/383;patch([0 1 1 0],[0 0 1 1],c1);patch([0 1 1 1-e 1-e 0+e],[0 0 1 1-e 0+e 0+e],c2);patch([0 0 1 1-e 0+e 0+e],[0 1 1 1-e 1-e 0+e],c3);plot([0 1 1 0 0],[0 0 1 1 0]);disp('weights');
  "IW{3,2}(8,:)'" : Constant  Value=[0.4825080990044359197099765879102051258087158203125;0.4454490793135317261430827784352004528045654296875;-0.309641435767183448302120041262242011725902557373046875;0.55067319427306238299735241525922901928424835205078125;0.5161985505789081773997395430342294275760650634765625;-0.30865473052762071315413550109951756894588470458984375;0.26353274705697771196355461142957210540771484375;-0.5759383149353585196195126627571880817413330078125;0.7056664845019937626346973047475330531597137451171875;-0.40892739841495429065076905317255295813083648681640625;-0.210971511522269838945220499226707033812999725341796875;0.74206406104037980764331905447761528193950653076171875;-0.33635595843181231856533486279658973217010498046875;-1.0256434728478966977860409315326251089572906494140625;-0.1120716899623792617290973794297315180301666259765625]
      mask Display: e = 0.06;c1 = [120 150 230]/255;c2 = ([120 150 230]+0)/383;c3 = ([120 150 230]+128)/383;patch([0 1 1 0],[0 0 1 1],c1);patch([0 1 1 1-e 1-e 0+e],[0 0 1 1-e 0+e 0+e],c2);patch([0 0 1 1-e 0+e 0+e],[0 1 1 1-e 1-e 0+e],c3);plot([0 1 1 0 0],[0 0 1 1 0]);disp('weights');
  "IW{3,2}(9,:)'" : Constant  Value=[-0.77083040673753921989685977678163908421993255615234375;-0.7792930387153027549373973670299164950847625732421875;0.324348642961859778832689471528283320367336273193359375;-0.7987873552751569850016721829888410866260528564453125;-0.1347153477057989601206600127625279128551483154296875;0.2197143385804321003007544277352280914783477783203125;-0.7470002693413941852185189418378286063671112060546875;-0.8453063837746463971001276149763725697994232177734375;-0.1956448615240838073692231091627036221325397491455078125;-0.1626434370914513483086238920805044472217559814453125;-0.53782366007346948943990128100267611443996429443359375;0.0331164167025408406885844669886864721775054931640625;-0.63852447949041124530822344240732491016387939453125;0.526717911604806854342086808173917233943939208984375;-0.8395538505272213125607549955020658671855926513671875]
      mask Display: e = 0.06;c1 = [120 150 230]/255;c2 = ([120 150 230]+0)/383;c3 = ([120 150 230]+128)/383;patch([0 1 1 0],[0 0 1 1],c1);patch([0 1 1 1-e 1-e 0+e],[0 0 1 1-e 0+e 0+e],c2);patch([0 0 1 1-e 0+e 0+e],[0 1 1 1-e 1-e 0+e],c3);plot([0 1 1 0 0],[0 0 1 1 0]);disp('weights');
  Mux : Mux  Inputs=15
      mask Display: e = 0.06;c1 = [120 150 230]/255;c2 = ([120 150 230]+0)/383;c3 = ([120 150 230]+128)/383;patch([0 1 1 0],[0 0 1 1],c1);patch([0 1 1 1-e 1-e 0+e],[0 0 1 1-e 0+e 0+e],c2);patch([0 0 1 1-e 0+e 0+e],[0 1 1 1-e 1-e 0+e],c3);plot([0 1 1 0 0],[0 0 1 1 0]);disp('Mux');
  dotprod{1..15} (15 alike) : neural/Weight Functions/dotprod
  "lz{3,2}" : Outport
      mask Display: e = 0.06;c1 = [120 230 180]/255;c2 = ([120 230 180]+0)/(256+128);c3 = ([120 230 180]+128)/(256+128);patch([0 1 1 0],[0 0 1 1],c1);patch([0 1 1 1-e 1-e 0+e],[0 0 1 1-e 0+e 0+e],c2);patch([0 0 1 1-e 0+e 0+e],[0 1 1 1-e 1-e 0+e],c3);plot([0 1 1 0 0],[0 0 1 1 0]);
  wires:
  Mux/1 -> "lz{3,2}"/1
  dotprod15/1 -> Mux/15
  "IW{3,2}(15,:)'"/1 -> dotprod15/1
  dotprod14/1 -> Mux/14
  "IW{3,2}(14,:)'"/1 -> dotprod14/1
  dotprod13/1 -> Mux/13
  "IW{3,2}(13,:)'"/1 -> dotprod13/1
  dotprod12/1 -> Mux/12
  "IW{3,2}(12,:)'"/1 -> dotprod12/1
  dotprod11/1 -> Mux/11
  "IW{3,2}(11,:)'"/1 -> dotprod11/1
  dotprod10/1 -> Mux/10
  "IW{3,2}(10,:)'"/1 -> dotprod10/1
  dotprod9/1 -> Mux/9
  "IW{3,2}(9,:)'"/1 -> dotprod9/1
  dotprod8/1 -> Mux/8
  "IW{3,2}(8,:)'"/1 -> dotprod8/1
  dotprod7/1 -> Mux/7
  "IW{3,2}(7,:)'"/1 -> dotprod7/1
  dotprod6/1 -> Mux/6
  "IW{3,2}(6,:)'"/1 -> dotprod6/1
  dotprod5/1 -> Mux/5
  "IW{3,2}(5,:)'"/1 -> dotprod5/1
  dotprod4/1 -> Mux/4
  "IW{3,2}(4,:)'"/1 -> dotprod4/1
  dotprod3/1 -> Mux/3
  "IW{3,2}(3,:)'"/1 -> dotprod3/1
  dotprod2/1 -> Mux/2
  "IW{3,2}(2,:)'"/1 -> dotprod2/1
  dotprod1/1 -> Mux/1
  "ad{3,2}"/1 -> dotprod15/2, dotprod14/2, dotprod13/2, dotprod12/2, dotprod11/2, dotprod10/2, dotprod9/2, dotprod8/2, dotprod7/2, dotprod6/2, dotprod5/2, dotprod4/2, dotprod3/2, dotprod2/2, dotprod1/2
  "IW{3,2}(1,:)'"/1 -> dotprod1/1

== system ACC4_FFNN_trainbfg_15_15_15_ep_100_Nor_20250527/Feed-Forward Neural Network/Layer 4/Delays 1 ==
  "p{4}" : Inport  PortDimensions=15
      mask Display: e = 0.06;c1 = [120 230 180]/255;c2 = ([120 230 180]+0)/(256+128);c3 = ([120 230 180]+128)/(256+128);patch([0 1 1 0],[0 0 1 1],c1);patch([0 1 1 1-e 1-e 0+e],[0 0 1 1-e 0+e 0+e],c2);patch([0 0 1 1-e 0+e 0+e],[0 1 1 1-e 1-e 0+e],c3);plot([0 1 1 0 0],[0 0 1 1 0]);
  mux : Mux  Inputs=1
      mask Display: e = 0.06;c1 = [120 150 230]/255;c2 = ([120 150 230]+0)/383;c3 = ([120 150 230]+128)/383;patch([0 1 1 0],[0 0 1 1],c1);patch([0 1 1 1-e 1-e 0+e],[0 0 1 1-e 0+e 0+e],c2);patch([0 0 1 1-e 0+e 0+e],[0 1 1 1-e 1-e 0+e],c3);plot([0 1 1 0 0],[0 0 1 1 0]);disp('Mux')
  "pd{4,3}" : Outport
      mask Display: e = 0.06;c1 = [120 230 180]/255;c2 = ([120 230 180]+0)/(256+128);c3 = ([120 230 180]+128)/(256+128);patch([0 1 1 0],[0 0 1 1],c1);patch([0 1 1 1-e 1-e 0+e],[0 0 1 1-e 0+e 0+e],c2);patch([0 0 1 1-e 0+e 0+e],[0 1 1 1-e 1-e 0+e],c3);plot([0 1 1 0 0],[0 0 1 1 0]);
  wires:
  mux/1 -> "pd{4,3}"/1
  "p{4}"/1 -> mux/1

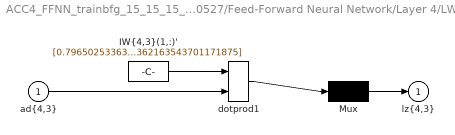
== system ACC4_FFNN_trainbfg_15_15_15_ep_100_Nor_20250527/Feed-Forward Neural Network/Layer 4/LW{4,3} ==
  "ad{4,3}" : Inport  PortDimensions=15
      mask Display: e = 0.06;c1 = [120 230 180]/255;c2 = ([120 230 180]+0)/(256+128);c3 = ([120 230 180]+128)/(256+128);patch([0 1 1 0],[0 0 1 1],c1);patch([0 1 1 1-e 1-e 0+e],[0 0 1 1-e 0+e 0+e],c2);patch([0 0 1 1-e 0+e 0+e],[0 1 1 1-e 1-e 0+e],c3);plot([0 1 1 0 0],[0 0 1 1 0]);
  "IW{4,3}(1,:)'" : Constant  Value=[0.79650253363963641195510945181013084948062896728515625;-0.2528723847147100745047509917640127241611480712890625;-0.431953372351024544872899468828109093010425567626953125;0.322629932680649156306884606237872503697872161865234375;-0.59495316788778118688441054473514668643474578857421875;-0.03843451082897442194763470979523845016956329345703125;0.43933801520293924713911337676108814775943756103515625;-0.0793832726429817003843680822683381848037242889404296875;-0.335789789829236073881446600353228859603404998779296875;-0.4016263107236024421098363745841197669506072998046875;0.1989991446802277519356749735379707999527454376220703125;-0.0123442011911747522023841128202548134140670299530029296875;0.91789250807903577378255022267694585025310516357421875;0.6011173125576221298871359977056272327899932861328125;0.5505047804119029830616227627615444362163543701171875]
      mask Display: e = 0.06;c1 = [120 150 230]/255;c2 = ([120 150 230]+0)/383;c3 = ([120 150 230]+128)/383;patch([0 1 1 0],[0 0 1 1],c1);patch([0 1 1 1-e 1-e 0+e],[0 0 1 1-e 0+e 0+e],c2);patch([0 0 1 1-e 0+e 0+e],[0 1 1 1-e 1-e 0+e],c3);plot([0 1 1 0 0],[0 0 1 1 0]);disp('weights');
  Mux : Mux  Inputs=1
      mask Display: e = 0.06;c1 = [120 150 230]/255;c2 = ([120 150 230]+0)/383;c3 = ([120 150 230]+128)/383;patch([0 1 1 0],[0 0 1 1],c1);patch([0 1 1 1-e 1-e 0+e],[0 0 1 1-e 0+e 0+e],c2);patch([0 0 1 1-e 0+e 0+e],[0 1 1 1-e 1-e 0+e],c3);plot([0 1 1 0 0],[0 0 1 1 0]);disp('Mux');
  dotprod1 : neural/Weight Functions/dotprod
  "lz{4,3}" : Outport
      mask Display: e = 0.06;c1 = [120 230 180]/255;c2 = ([120 230 180]+0)/(256+128);c3 = ([120 230 180]+128)/(256+128);patch([0 1 1 0],[0 0 1 1],c1);patch([0 1 1 1-e 1-e 0+e],[0 0 1 1-e 0+e 0+e],c2);patch([0 0 1 1-e 0+e 0+e],[0 1 1 1-e 1-e 0+e],c3);plot([0 1 1 0 0],[0 0 1 1 0]);
  wires:
  Mux/1 -> "lz{4,3}"/1
  dotprod1/1 -> Mux/1
  "ad{4,3}"/1 -> dotprod1/2
  "IW{4,3}(1,:)'"/1 -> dotprod1/1
